simulink model "tanker_cosim"  (R2022a)
settings: Solver=ode4  StartTime=0.0  StopTime=25  FixedStep=0.001  RelTol=1e-3
settings Model: Creator=LENOVO  LastModifiedBy=LENOVO

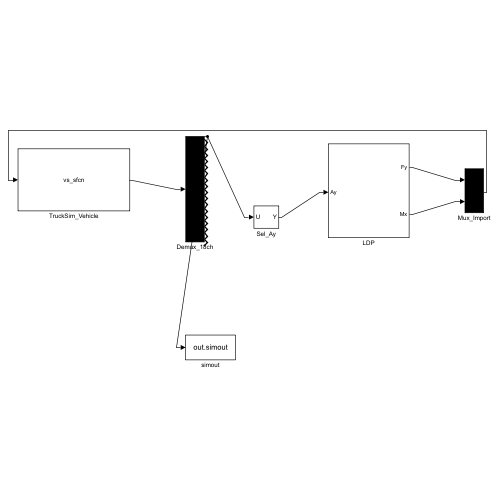
[thumbnail: Simulink's stored preview of the top-level diagram]
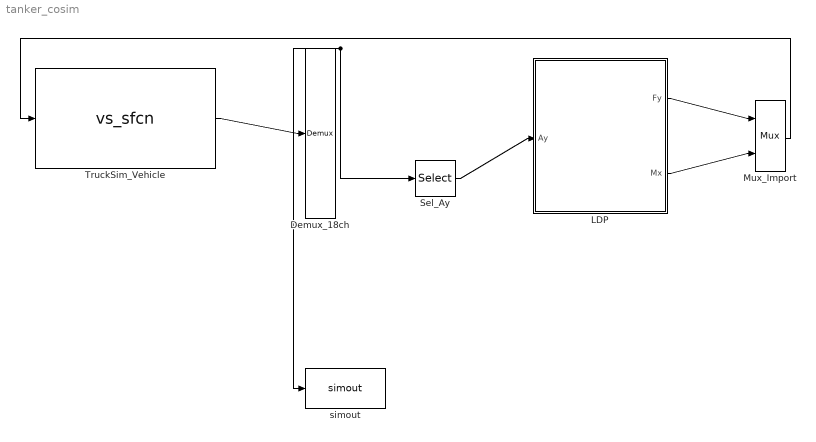
== system tanker_cosim ==
  Demux_18ch : Demux  Outputs=18
  LDP : Subsystem
  Mux_Import : Mux  Inputs=2
  Sel_Ay : Selector  InputPortWidth=18  IndexOptions=Index vector (dialog)  Indices=2  OutputSizes=1
  TruckSim_Vehicle : S-Function  FunctionName=vs_sfcn  SFunctionDeploymentMode=off  EnableBusSupport=off
  simout : ToWorkspace  VariableName=simout  SaveFormat=Structure With Time  SampleTime=-1
  wires:
  TruckSim_Vehicle/1 -> Demux_18ch/1
  Demux_18ch/1 -> Sel_Ay/1, simout/1
  Sel_Ay/1 -> LDP/1(Ay)
  LDP/1(Fy) -> Mux_Import/1
  LDP/2(Mx) -> Mux_Import/2
  Mux_Import/1 -> TruckSim_Vehicle/1

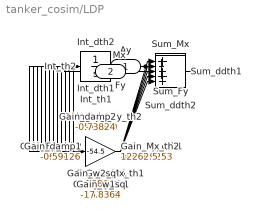
== system tanker_cosim/LDP ==
  Ay : Inport
  Gain_Ay_L1 : Gain  Gain=-1.8182
  Gain_Ay_L2 : Gain  Gain=-5.5556
  Gain_Fy_dth1 : Gain  Gain=-4877.9253
  Gain_Fy_dth2 : Gain  Gain=-664.417
  Gain_Fy_th1 : Gain  Gain=-147150
  Gain_Fy_th2 : Gain  Gain=-49050
  Gain_Mx_th1 : Gain  Gain=58860
  Gain_Mx_th2 : Gain  Gain=12262.5
  Gain_damp1 : Gain  Gain=-0.59126
  Gain_damp2 : Gain  Gain=-0.73824
  Gain_w1sq : Gain  Gain=-17.8364
  Gain_w2sq : Gain  Gain=-54.5
  Int_dth1 : Integrator
  Int_dth2 : Integrator
  Int_th1 : Integrator
  Int_th2 : Integrator
  Sum_Fy : Sum  Inputs=++++
  Sum_Mx : Sum
  Sum_ddth1 : Sum  Inputs=+++
  Sum_ddth2 : Sum  Inputs=+++
  Fy : Outport
  Mx : Outport  Port=2
  wires:
  ? -> ?
  Ay/1 -> Gain_Ay_L1/1, Gain_Ay_L2/1
  Int_th1/1 -> Gain_w1sq/1, Gain_Fy_th1/1, Gain_Mx_th1/1
  Int_dth1/1 -> Gain_damp1/1, Int_th1/1, Gain_Fy_dth1/1
  Gain_Ay_L1/1 -> Sum_ddth1/1
  Gain_w1sq/1 -> Sum_ddth1/2
  Gain_damp1/1 -> Sum_ddth1/3
  Sum_ddth1/1 -> Int_dth1/1
  Int_th2/1 -> Gain_w2sq/1, Gain_Fy_th2/1, Gain_Mx_th2/1
  Int_dth2/1 -> Gain_damp2/1, Int_th2/1, Gain_Fy_dth2/1
  Gain_Ay_L2/1 -> Sum_ddth2/1
  Gain_w2sq/1 -> Sum_ddth2/2
  Gain_damp2/1 -> Sum_ddth2/3
  Sum_ddth2/1 -> Int_dth2/1
  Gain_Fy_th1/1 -> Sum_Fy/1
  Gain_Fy_dth1/1 -> Sum_Fy/2
  Gain_Fy_th2/1 -> Sum_Fy/3
  Gain_Fy_dth2/1 -> Sum_Fy/4
  Sum_Fy/1 -> Fy/1
  Gain_Mx_th1/1 -> Sum_Mx/1
  Gain_Mx_th2/1 -> Sum_Mx/2
  Sum_Mx/1 -> Mx/1
